simulink model "w6_stage4_4_thermal_cooling"  (R2026a)
settings: Solver=ode45  StopTime=600  MaxStep=0.1  RelTol=1e-10  AbsTol=1e-12
settings Model: Creator=cogml  LastModifiedBy=cogml

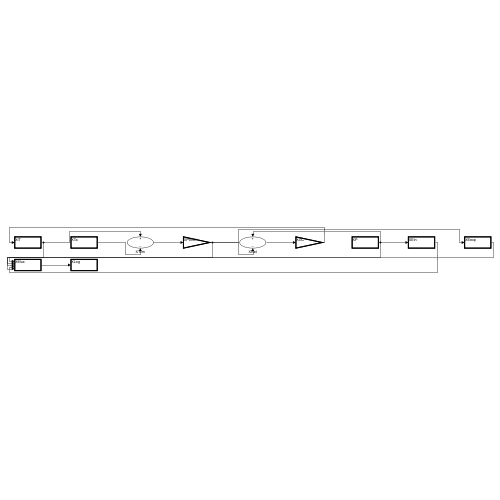
[thumbnail: Simulink's stored preview of the top-level diagram]
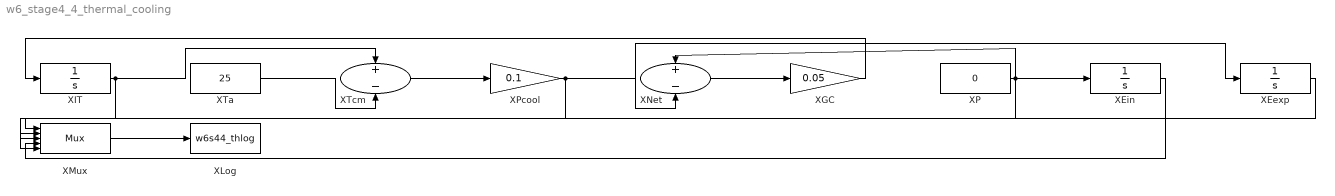
== system w6_stage4_4_thermal_cooling ==
  XEexp : Integrator
  XEin : Integrator
  XGC : Gain  Gain=0.05
  XIT : Integrator  InitialCondition=80
  XLog : ToWorkspace  VariableName=w6s44_thlog  SaveFormat=Timeseries  SampleTime=0.1
  XMux : Mux  Inputs=5
  XNet : Sum  Inputs=+-
  XP : Constant  Value=0
  XPcool : Gain  Gain=0.1
  XTa : Constant  Value=25
  XTcm : Sum  Inputs=+-
  wires:
  XIT/1 -> XTcm/1, XMux/1
  XTa/1 -> XTcm/2
  XTcm/1 -> XPcool/1
  XNet/1 -> XGC/1
  XGC/1 -> XIT/1
  XPcool/1 -> XNet/2, XEexp/1, XMux/3
  XP/1 -> XNet/1, XEin/1, XMux/2
  XEin/1 -> XMux/4
  XEexp/1 -> XMux/5
  XMux/1 -> XLog/1
